simulink model "Non_Linear_Model"  (R2024b)
settings: Solver=VariableStepAuto  StartTime=0.0  StopTime=10  RelTol=1e-5
values from neighbouring files (symbols this model uses):
  Ca_f = 125000    [vehicle_var.m]
  Ca_r = 80000    [vehicle_var.m]
  eta = 0.15    [vehicle_var.m]
  I = 1500    [vehicle_var.m]
  K_inf = [-0.162, -0.895, -9.794, -1.394]    [vehicle_var.m]
  lf = 0.92    [vehicle_var.m]
  lr = 1.38    [vehicle_var.m]
  M = 1200    [vehicle_var.m]
  vx = 22    [vehicle_var.m]
libraries: simulink x6
settings Model: Creator=Antonio  LastModifiedBy=Antonio

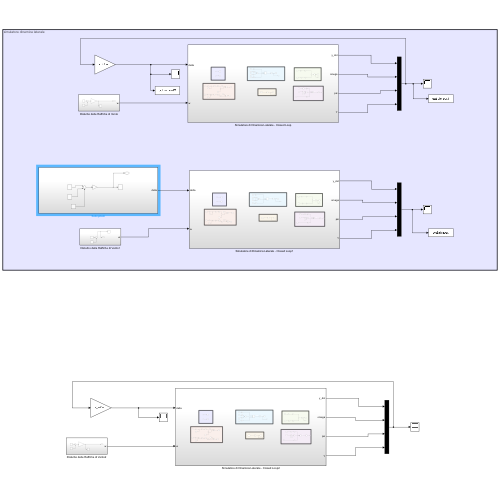
[thumbnail: Simulink's stored preview of the top-level diagram]
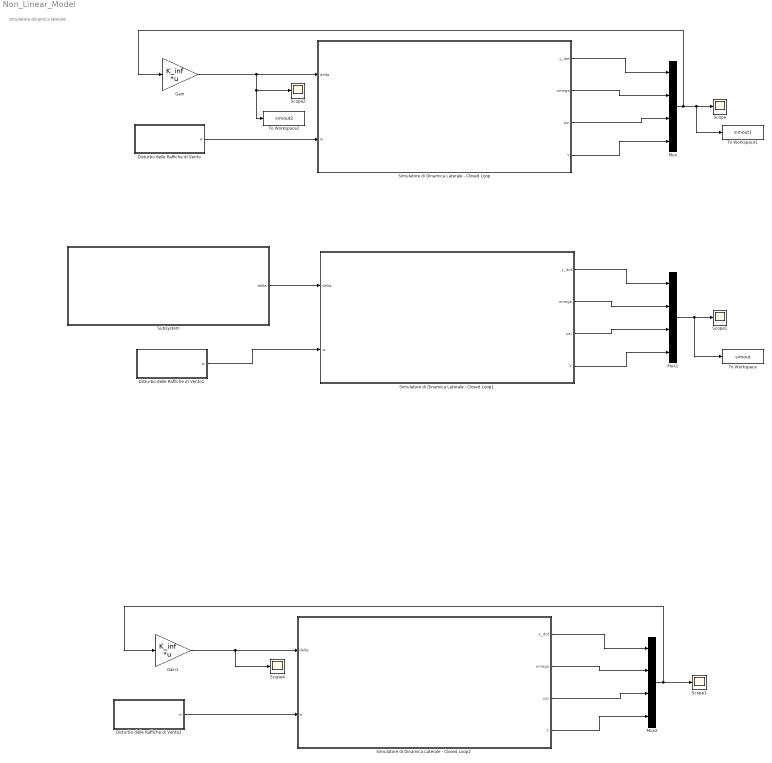
== system Non_Linear_Model ==
  note: simulatore dinamica laterale
  Disturbo delle Raffiche di Vento : Subsystem
  Disturbo delle Raffiche di Vento1 : Subsystem
  Disturbo delle Raffiche di Vento2 : Subsystem
  Gain : Gain  Gain=K_inf  Multiplication=Matrix(K*u)
  Gain1 : Gain  Gain=K_inf  Multiplication=Matrix(K*u)
  Mux : Mux
  Mux1 : Mux
  Mux2 : Mux
  Scope{,1..4} (5 alike) : Scope
  Simulatore di Dinamica Laterale - Closed Loop : Subsystem
  Simulatore di Dinamica Laterale - Closed Loop1 : Subsystem
  Simulatore di Dinamica Laterale - Closed Loop2 : Subsystem
  Subsystem : Subsystem
  To Workspace : ToWorkspace  VariableName=simout  SaveFormat=Timeseries  SampleTime=-1
  To Workspace1 : ToWorkspace  VariableName=simout1  SaveFormat=Timeseries  SampleTime=-1
  To Workspace2 : ToWorkspace  VariableName=simout2  SaveFormat=Timeseries  SampleTime=-1
  wires:
  Simulatore di Dinamica Laterale - Closed Loop1/3(psi) -> Mux1/3
  Simulatore di Dinamica Laterale - Closed Loop1/2(omega) -> Mux1/2
  Simulatore di Dinamica Laterale - Closed Loop1/4(Y) -> Mux1/4
  Simulatore di Dinamica Laterale - Closed Loop1/1(y_dot) -> Mux1/1
  Mux1/1 -> To Workspace/1, Scope1/1
  Mux/1 -> Gain/1, To Workspace1/1, Scope/1
  Disturbo delle Raffiche di Vento/1(w) -> Simulatore di Dinamica Laterale - Closed Loop/2(w)
  Simulatore di Dinamica Laterale - Closed Loop/3(psi) -> Mux/3
  Simulatore di Dinamica Laterale - Closed Loop/1(y_dot) -> Mux/1
  Simulatore di Dinamica Laterale - Closed Loop/4(Y) -> Mux/4
  Simulatore di Dinamica Laterale - Closed Loop/2(omega) -> Mux/2
  Subsystem/1(delta) -> Simulatore di Dinamica Laterale - Closed Loop1/1(delta)
  Disturbo delle Raffiche di Vento1/1(w) -> Simulatore di Dinamica Laterale - Closed Loop1/2(w)
  Gain/1 -> Simulatore di Dinamica Laterale - Closed Loop/1(delta), To Workspace2/1, Scope2/1
  Disturbo delle Raffiche di Vento2/1(w) -> Simulatore di Dinamica Laterale - Closed Loop2/2(w)
  Mux2/1 -> Gain1/1, Scope3/1
  Simulatore di Dinamica Laterale - Closed Loop2/2(omega) -> Mux2/2
  Gain1/1 -> Simulatore di Dinamica Laterale - Closed Loop2/1(delta), Scope4/1
  Simulatore di Dinamica Laterale - Closed Loop2/4(Y) -> Mux2/4
  Simulatore di Dinamica Laterale - Closed Loop2/3(psi) -> Mux2/3
  Simulatore di Dinamica Laterale - Closed Loop2/1(y_dot) -> Mux2/1

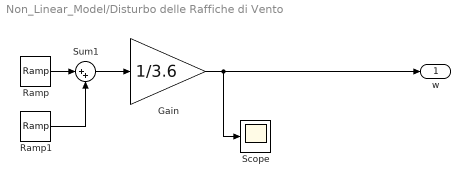
== system Non_Linear_Model/Disturbo delle Raffiche di Vento ==
  Gain : Gain  Gain=1/3.6
  Ramp : simulink/Sources/Ramp  slope=-8  start=2  InitialOutput=0
  Ramp1 : simulink/Sources/Ramp  slope=8  start=3  InitialOutput=9
  Scope : Scope
  Sum1 : Sum  Inputs=|++
  w : Outport
  wires:
  Ramp/1 -> Sum1/1
  Ramp1/1 -> Sum1/2
  Sum1/1 -> Gain/1
  Gain/1 -> Scope/1, w/1

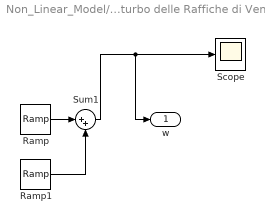
== system Non_Linear_Model/Disturbo delle Raffiche di Vento1 ==
  Ramp : simulink/Sources/Ramp  slope=-8  start=2  InitialOutput=0
  Ramp1 : simulink/Sources/Ramp  slope=8  start=3  InitialOutput=9
  Scope : Scope
  Sum1 : Sum  Inputs=|++
  w : Outport
  wires:
  Ramp/1 -> Sum1/1
  Sum1/1 -> w/1, Scope/1
  Ramp1/1 -> Sum1/2

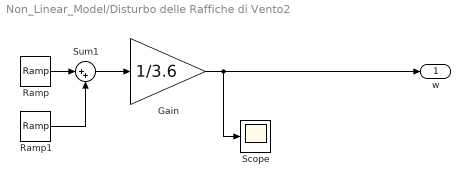
== system Non_Linear_Model/Disturbo delle Raffiche di Vento2 ==
  Gain : Gain  Gain=1/3.6
  Ramp : simulink/Sources/Ramp  slope=-8  start=2  InitialOutput=0
  Ramp1 : simulink/Sources/Ramp  slope=8  start=3  InitialOutput=9
  Scope : Scope
  Sum1 : Sum  Inputs=|++
  w : Outport
  wires:
  Ramp/1 -> Sum1/1
  Ramp1/1 -> Sum1/2
  Sum1/1 -> Gain/1
  Gain/1 -> Scope/1, w/1

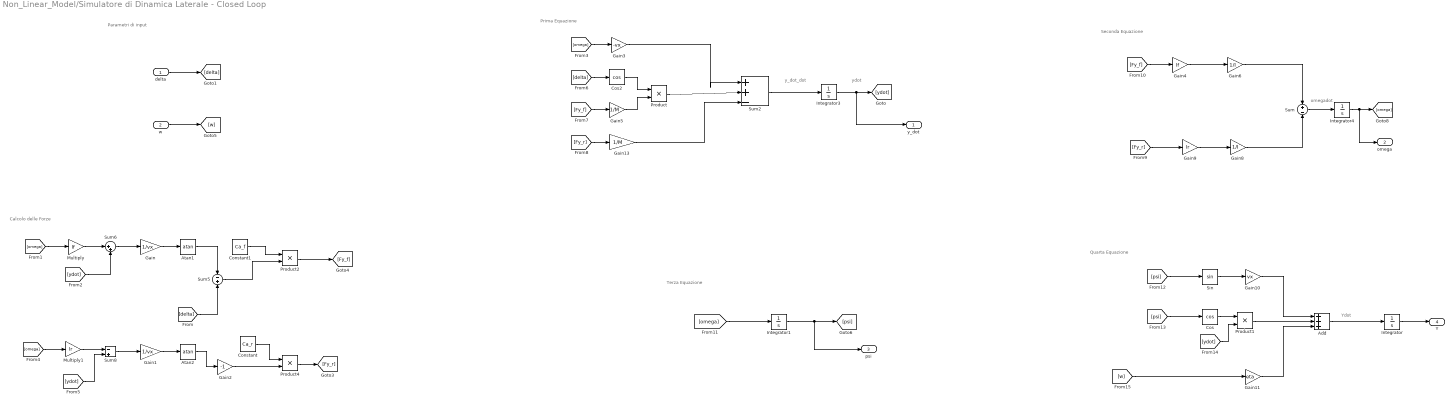
== system Non_Linear_Model/Simulatore di Dinamica Laterale - Closed Loop ==
  note: Ydot
  note: Quarta Equazione
  note: Terza Equazione
  note: omegadot
  note: Seconda Equazione
  note: Prima Equazione
  note: Calcolo delle Forze
  note: Parametri di input
  note: ydot
  note: y_dot_dot
  delta : Inport
  w : Inport  Port=2
  Add : Sum  Inputs=+++
  Atan1 : Trigonometry  Operator=atan
  Atan2 : Trigonometry  Operator=atan
  Constant : Constant  Value=Ca_r
  Constant1 : Constant  Value=Ca_f
  Cos : Trigonometry  Operator=cos
  Cos2 : Trigonometry  Operator=cos
  Gain : Gain  Gain=1/vx
  Gain1 : Gain  Gain=1/vx
  Gain10 : Gain  Gain=vx
  Gain11 : Gain  Gain=eta
  Gain13 : Gain  Gain=1/M
  Gain2 : Gain  Gain=-1
  Gain3 : Gain  Gain=-vx
  Gain4 : Gain  Gain=lf
  Gain5 : Gain  Gain=1/M
  Gain6 : Gain  Gain=1/I
  Gain8 : Gain  Gain=1/I
  Gain9 : Gain  Gain=lr
  Integrator{,1,3..4} (4 alike) : Integrator
  Multiply : Gain  Gain=lf
  Multiply1 : Gain  Gain=lr
  Product{,1..2,4} (4 alike) : Product
  Sin : Trigonometry
  Sum : Sum  Inputs=+|-
  Sum2 : Sum  Inputs=|++-
  Sum5 : Sum  Inputs=-|+
  Sum6 : Sum  Inputs=|++
  Sum8 : Sum  Inputs=-|+
  y_dot : Outport
  omega : Outport  Port=2
  psi : Outport  Port=3
  Y : Outport  Port=4
  wires:
  Multiply/1 -> Sum6/1
  [delta] -> Sum5/2
  [omega] -> Integrator1/1
  Gain2/1 -> Product4/2
  Cos/1 -> Product1/1
  [Fy_r] -> Gain13/1
  Product/1 -> Sum2/2
  Integrator4/1 -> omega/1, [omega]
  [Fy_f] -> Gain5/1
  [ydot] -> Sum6/2
  Gain1/1 -> Atan2/1
  Gain4/1 -> Gain6/1
  Sum/1 -> Integrator4/1
  [delta] -> Cos2/1
  Gain11/1 -> Add/3
  Gain/1 -> Atan1/1
  [w] -> Gain11/1
  Gain8/1 -> Sum/2
  Integrator3/1 -> y_dot/1, [ydot]
  Cos2/1 -> Product/1
  Gain6/1 -> Sum/1
  Sum8/1 -> Gain1/1
  [omega] -> Multiply1/1
  delta/1 -> [delta]
  Multiply1/1 -> Sum8/1
  [ydot] -> Product1/2
  Gain9/1 -> Gain8/1
  Gain5/1 -> Product/2
  [Fy_r] -> Gain9/1
  Sum6/1 -> Gain/1
  [ydot] -> Sum8/2
  Atan2/1 -> Gain2/1
  Gain13/1 -> Sum2/3
  Product1/1 -> Add/2
  Atan1/1 -> Sum5/1
  Gain3/1 -> Sum2/1
  [omega] -> Gain3/1
  [psi] -> Sin/1
  Integrator1/1 -> psi/1, [psi]
  Add/1 -> Integrator/1
  Gain10/1 -> Add/1
  [omega] -> Multiply/1
  Sin/1 -> Gain10/1
  Integrator/1 -> Y/1
  [psi] -> Cos/1
  Sum5/1 -> Product2/2
  w/1 -> [w]
  Sum2/1 -> Integrator3/1
  [Fy_f] -> Gain4/1
  Product4/1 -> [Fy_r]
  Product2/1 -> [Fy_f]
  Constant/1 -> Product4/1
  Constant1/1 -> Product2/1

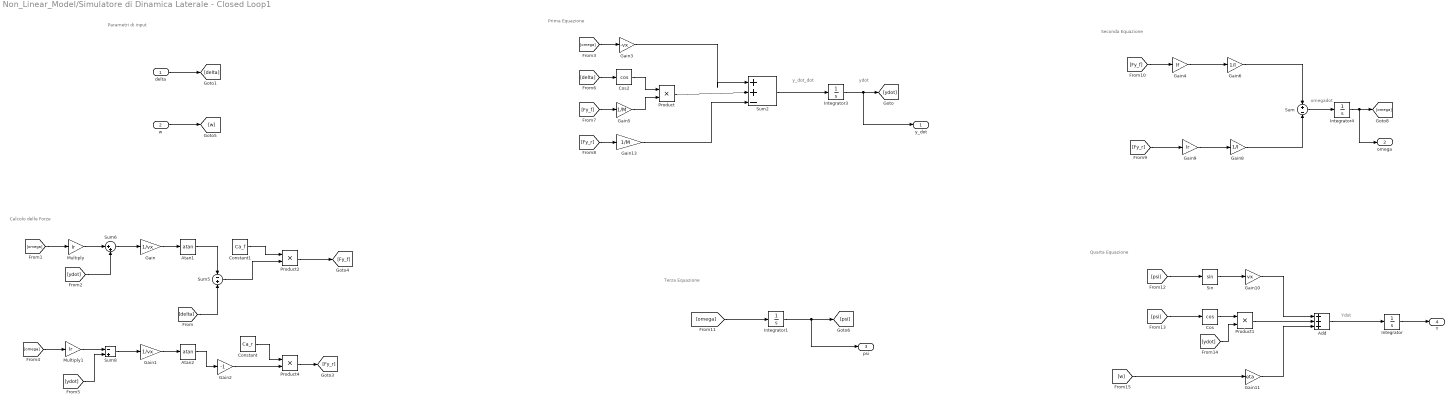
== system Non_Linear_Model/Simulatore di Dinamica Laterale - Closed Loop1 ==
  note: Ydot
  note: Quarta Equazione
  note: Terza Equazione
  note: omegadot
  note: Seconda Equazione
  note: Prima Equazione
  note: Calcolo delle Forze
  note: Parametri di input
  note: ydot
  note: y_dot_dot
  delta : Inport
  w : Inport  Port=2
  Add : Sum  Inputs=+++
  Atan1 : Trigonometry  Operator=atan
  Atan2 : Trigonometry  Operator=atan
  Constant : Constant  Value=Ca_r
  Constant1 : Constant  Value=Ca_f
  Cos : Trigonometry  Operator=cos
  Cos2 : Trigonometry  Operator=cos
  Gain : Gain  Gain=1/vx
  Gain1 : Gain  Gain=1/vx
  Gain10 : Gain  Gain=vx
  Gain11 : Gain  Gain=eta
  Gain13 : Gain  Gain=1/M
  Gain2 : Gain  Gain=-1
  Gain3 : Gain  Gain=-vx
  Gain4 : Gain  Gain=lf
  Gain5 : Gain  Gain=1/M
  Gain6 : Gain  Gain=1/I
  Gain8 : Gain  Gain=1/I
  Gain9 : Gain  Gain=lr
  Integrator{,1,3..4} (4 alike) : Integrator
  Multiply : Gain  Gain=lr
  Multiply1 : Gain  Gain=lr
  Product{,1..2,4} (4 alike) : Product
  Sin : Trigonometry
  Sum : Sum  Inputs=+|-
  Sum2 : Sum  Inputs=|++-
  Sum5 : Sum  Inputs=-|+
  Sum6 : Sum  Inputs=|++
  Sum8 : Sum  Inputs=-|+
  y_dot : Outport
  omega : Outport  Port=2
  psi : Outport  Port=3
  Y : Outport  Port=4
  wires:
  Multiply/1 -> Sum6/1
  [delta] -> Sum5/2
  [omega] -> Integrator1/1
  Gain2/1 -> Product4/2
  Cos/1 -> Product1/1
  [Fy_r] -> Gain13/1
  Product/1 -> Sum2/2
  Integrator4/1 -> omega/1, [omega]
  [Fy_f] -> Gain5/1
  [ydot] -> Sum6/2
  Gain1/1 -> Atan2/1
  Gain4/1 -> Gain6/1
  Sum/1 -> Integrator4/1
  [delta] -> Cos2/1
  Gain11/1 -> Add/3
  Gain/1 -> Atan1/1
  [w] -> Gain11/1
  Gain8/1 -> Sum/2
  Integrator3/1 -> y_dot/1, [ydot]
  Cos2/1 -> Product/1
  Gain6/1 -> Sum/1
  Sum8/1 -> Gain1/1
  [omega] -> Multiply1/1
  delta/1 -> [delta]
  Multiply1/1 -> Sum8/1
  [ydot] -> Product1/2
  Gain9/1 -> Gain8/1
  Gain5/1 -> Product/2
  [Fy_r] -> Gain9/1
  Sum6/1 -> Gain/1
  [ydot] -> Sum8/2
  Atan2/1 -> Gain2/1
  Gain13/1 -> Sum2/3
  Product1/1 -> Add/2
  Atan1/1 -> Sum5/1
  Gain3/1 -> Sum2/1
  [omega] -> Gain3/1
  [psi] -> Sin/1
  Integrator1/1 -> psi/1, [psi]
  Add/1 -> Integrator/1
  Gain10/1 -> Add/1
  [omega] -> Multiply/1
  Sin/1 -> Gain10/1
  Integrator/1 -> Y/1
  [psi] -> Cos/1
  Sum5/1 -> Product2/2
  w/1 -> [w]
  Sum2/1 -> Integrator3/1
  [Fy_f] -> Gain4/1
  Product4/1 -> [Fy_r]
  Product2/1 -> [Fy_f]
  Constant/1 -> Product4/1
  Constant1/1 -> Product2/1

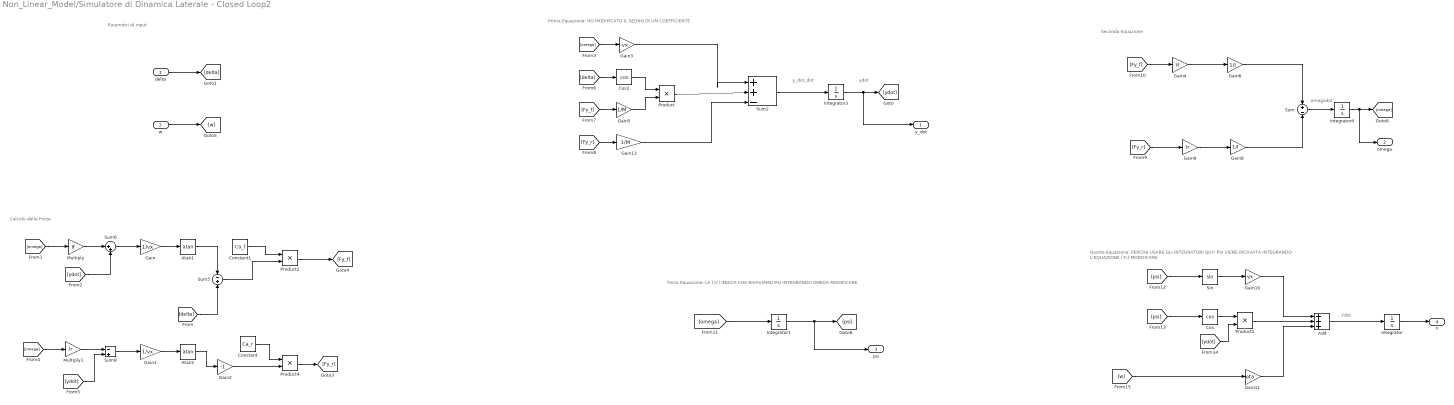
== system Non_Linear_Model/Simulatore di Dinamica Laterale - Closed Loop2 ==
  note: Ydot
  note: Quarta Equazione: PERCHè USARE GLI INTEGRATORI QUI? PSI VIENE RICAVATA INTEGRANDO L'EQUAZIONE (7c)
      | MODIFICARE
  note: Terza Equazione: LA (7c) INDICA CHE RIVAVIAMO PSI INTEGRANDO OMEGA
      | MODIFICARE
  note: omegadot
  note: Seconda Equazione
  note: Prima Equazione: HO MODIFICATO IL SEGNO DI UN COEFFICIENTE
  note: Calcolo delle Forze
  note: Parametri di input
  note: ydot
  note: y_dot_dot
  delta : Inport
  w : Inport  Port=2
  Add : Sum  Inputs=+++
  Atan1 : Trigonometry  Operator=atan
  Atan2 : Trigonometry  Operator=atan
  Constant : Constant  Value=Ca_r
  Constant1 : Constant  Value=Ca_f
  Cos : Trigonometry  Operator=cos
  Cos2 : Trigonometry  Operator=cos
  Gain : Gain  Gain=1/vx
  Gain1 : Gain  Gain=1/vx
  Gain10 : Gain  Gain=vx
  Gain11 : Gain  Gain=eta
  Gain13 : Gain  Gain=1/M
  Gain2 : Gain  Gain=-1
  Gain3 : Gain  Gain=-vx
  Gain4 : Gain  Gain=lf
  Gain5 : Gain  Gain=1/M
  Gain6 : Gain  Gain=1/I
  Gain8 : Gain  Gain=1/I
  Gain9 : Gain  Gain=lr
  Integrator{,1,3..4} (4 alike) : Integrator
  Multiply : Gain  Gain=lf
  Multiply1 : Gain  Gain=lr
  Product{,1..2,4} (4 alike) : Product
  Sin : Trigonometry
  Sum : Sum  Inputs=+|-
  Sum2 : Sum  Inputs=|++-
  Sum5 : Sum  Inputs=-|+
  Sum6 : Sum  Inputs=|++
  Sum8 : Sum  Inputs=-|+
  y_dot : Outport
  omega : Outport  Port=2
  psi : Outport  Port=3
  Y : Outport  Port=4
  wires:
  Multiply/1 -> Sum6/1
  [delta] -> Sum5/2
  [omega] -> Integrator1/1
  Gain2/1 -> Product4/2
  Cos/1 -> Product1/1
  [Fy_r] -> Gain13/1
  Product/1 -> Sum2/2
  Integrator4/1 -> omega/1, [omega]
  [Fy_f] -> Gain5/1
  [ydot] -> Sum6/2
  Gain1/1 -> Atan2/1
  Gain4/1 -> Gain6/1
  Sum/1 -> Integrator4/1
  [delta] -> Cos2/1
  Gain11/1 -> Add/3
  Gain/1 -> Atan1/1
  [w] -> Gain11/1
  Gain8/1 -> Sum/2
  Integrator3/1 -> y_dot/1, [ydot]
  Cos2/1 -> Product/1
  Gain6/1 -> Sum/1
  Sum8/1 -> Gain1/1
  [omega] -> Multiply1/1
  delta/1 -> [delta]
  Multiply1/1 -> Sum8/1
  [ydot] -> Product1/2
  Gain9/1 -> Gain8/1
  Gain5/1 -> Product/2
  [Fy_r] -> Gain9/1
  Sum6/1 -> Gain/1
  [ydot] -> Sum8/2
  Atan2/1 -> Gain2/1
  Gain13/1 -> Sum2/3
  Product1/1 -> Add/2
  Atan1/1 -> Sum5/1
  Gain3/1 -> Sum2/1
  [omega] -> Gain3/1
  [psi] -> Sin/1
  Integrator1/1 -> psi/1, [psi]
  Add/1 -> Integrator/1
  Gain10/1 -> Add/1
  [omega] -> Multiply/1
  Sin/1 -> Gain10/1
  Integrator/1 -> Y/1
  [psi] -> Cos/1
  Sum5/1 -> Product2/2
  w/1 -> [w]
  Sum2/1 -> Integrator3/1
  [Fy_f] -> Gain4/1
  Product4/1 -> [Fy_r]
  Product2/1 -> [Fy_f]
  Constant/1 -> Product4/1
  Constant1/1 -> Product2/1

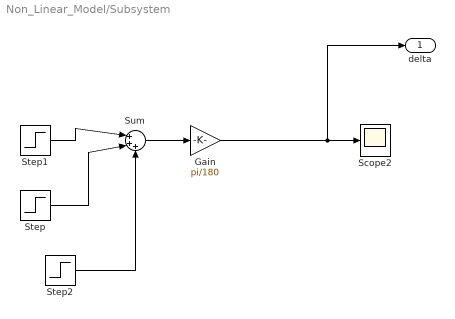
== system Non_Linear_Model/Subsystem ==
  Gain : Gain  Gain=pi/180
  Scope2 : Scope
  Step : Step  Time=4  After=-2  SampleTime=0
  Step1 : Step  Time=2  SampleTime=0
  Step2 : Step  Time=6  SampleTime=0
  Sum : Sum  Inputs=|+++
  delta : Outport
  wires:
  Sum/1 -> Gain/1
  Step1/1 -> Sum/1
  Gain/1 -> delta/1, Scope2/1
  Step/1 -> Sum/2
  Step2/1 -> Sum/3
